simulink model "classic_dtc_final"  (R2026a)
settings: Solver=VariableStepAuto  StopTime=Tsim  MaxStep=1e-6
undefined symbols (not defined in the file): HB_lambda, HB_torque, J, Ki_speed, Kp_speed, lambda_ref, p, Rs, t_load, TL, TL_init, Ts_dtc, Vdc
libraries: nesl_utility x13, fl_lib x10, ee_lib x5, slpidlib x1
settings Model: Creator=kunal  LastModifiedBy=kunal
settings SimscapeCC: SimscapeLogType=none

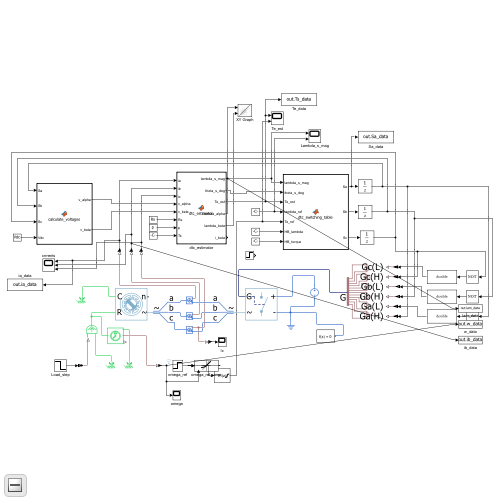
[thumbnail: Simulink's stored preview of the top-level diagram]
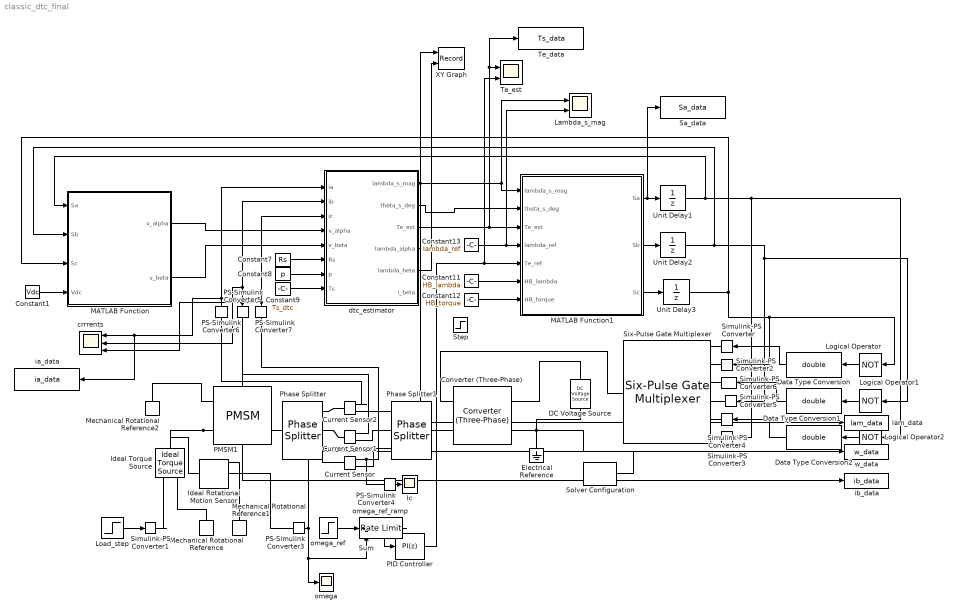
== system classic_dtc_final ==
  Constant1 : Constant  Value=Vdc
  Constant11 : Constant  Value=HB_lambda
  Constant12 : Constant  Value=HB_torque
  Constant13 : Constant  Value=lambda_ref
  Constant7 : Constant  Value=Rs
  Constant8 : Constant  Value=p
  Constant9 : Constant  Value=Ts_dtc
  Converter (Three-Phase) : ee_lib/Semiconductors & Converters/Converters/Converter (Three-Phase)  port_option=ee.enum.threePhasePort.composite  fidelity_option=ee.enum.converters.fidelity.detailed  device_type=ee.enum.converters.switchingdevice.ideal  showThermalPort=false  K=0  Vth=0.5 V  Vgt=1 V  Vgt_off=-1 V  Ih=1 A  Vf=0.8 V  Ron=0.001 Ohm  Rds=0.001 Ohm  Goff=1e-6 1/Ohm  Eon_scalar=22.86e-3 J  Eoff_scalar=17.14e-3 J  Eoff_natural_commutation=10e-3 J  Voff=300 V  Iout_scalar=600 A  onCurrentMeasDelay=0 s  useCurrentFromPreviousCycle=false  useVoltageFromPreviousCycle=false  diode_param=ee.enum.converters.protectiondiode.nodynamics  diode_Vf=0.8 V  diode_Ron=0.001 Ohm  diode_Goff=1e-5 1/Ohm  diode_C=50 nF  diode_iRM=-235 A  diode_iF=300 A  diode_idot=-50 A/us  diode_trr_param=ee.enum.converters.diodetrr.trr_factor  diode_trr_factor=3  diode_trr=15 us  diode_Qrr=1500 s*uA  diode_rec_loss_model=ee.enum.diode.reverseRecoveryModel.fixed  diode_ErecVal=0 J  diode_scaleWithIandV=false  diode_ErecMat=zeros(2, 3) J  diode_TjrecVec=[298.15, 398.15] K  diode_IfrecVec=[.1, 1, 10] A  diode_IrecVal=10 A  diode_VrecVal=10 V  diode_tFilter=1 / 1000 / 100 s  thermal_network_parameterization=ee.enum.thermalNetworkTopology.external  Rth=[.08, .5] K/W  Rth_Cauer=[.08, .1, .5] K/W  Rth_Foster=[.08, .14, .22, .16] K/W  thermal_mass_parameterization=ee.enum.thermalNetwork.timeconstant  thermal_mass=[.01, .5] J/K  thermal_mass_Cauer=[.01, .1, .5] J/K  thermal_mass_Foster=[.001, .005, .05, .5] J/K  thermal_time_constant=[.001, .2] s  thermal_time_constant_Cauer=[.001, .1, .2] s  thermal_time_constant_Foster=[7e-05, .0007, .01, .08] s  thermal_mass_initial_temperatures=[25, 25] degC  thermal_mass_initial_temperatures_Cauer=[25, 25, 25] degC  junction_thermal_mass=0.01 J/K  Tvec_initial_Foster=[25, 25, 25, 25] degC  snubber_type=ee.enum.converters.snubber.exclude  Cs=1e-7 F  Rs=0.1 Ohm  Vce_loss=[0, 150, 300] V
  Current Sensor : fl_lib/Electrical/Electrical Sensors/Current Sensor
  Current Sensor1 : fl_lib/Electrical/Electrical Sensors/Current Sensor
  Current Sensor2 : fl_lib/Electrical/Electrical Sensors/Current Sensor
  DC Voltage Source : fl_lib/Electrical/Electrical Sources/DC Voltage Source  v0=Vdc V
  Data Type Conversion : DataTypeConversion  OutDataTypeStr=double  SaturateOnIntegerOverflow=off  RndMeth=Floor
  Data Type Conversion1 : DataTypeConversion  OutDataTypeStr=double  SaturateOnIntegerOverflow=off  RndMeth=Floor
  Data Type Conversion2 : DataTypeConversion  OutDataTypeStr=double  SaturateOnIntegerOverflow=off  RndMeth=Floor
  Electrical Reference : fl_lib/Electrical/Electrical Elements/Electrical Reference
  Ic : Scope
      settings: ActiveDisplayYMinimum=-1.574268599657235  ActiveDisplayYMaximum=1.0954007787431075  DataLoggingVariableName=ScopeData3
  Ideal Rotational Motion Sensor : fl_lib/Mechanical/Mechanical Sensors/Ideal Rotational Motion Sensor  reference=foundation.enum.MeasurementReference.difference  acceleration_port=false  velocity_port=true  position_port=true  wrap_angle=false  offset=0 rad
  Ideal Torque Source : fl_lib/Mechanical/Mechanical Sources/Ideal Torque Source
  Lambda_s_mag : Scope  NumInputPorts=2
      settings: ActiveDisplayYMinimum=0.17238629365269534  ActiveDisplayYMaximum=0.17761260298821638
  Load_step : Step  Time=t_load  InitialValue=-TL_init  FinalValue=-TL  SampleTime=0
  Logical Operator : Logic  Operator=NOT  AllPortsSameDT=off  OutDataTypeStr=boolean
  Logical Operator1 : Logic  Operator=NOT  AllPortsSameDT=off  OutDataTypeStr=boolean
  Logical Operator2 : Logic  Operator=NOT  AllPortsSameDT=off  OutDataTypeStr=boolean
  MATLAB Function : MATLAB Function  TreatAsAtomicUnit=on  SystemSampleTime=Ts_dtc
  MATLAB Function1 : MATLAB Function  TreatAsAtomicUnit=on  SystemSampleTime=Ts_dtc
  Mechanical Rotational Reference : fl_lib/Mechanical/Rotational Elements/Mechanical Rotational Reference
  Mechanical Rotational Reference1 : fl_lib/Mechanical/Rotational Elements/Mechanical Rotational Reference
  Mechanical Rotational Reference2 : fl_lib/Mechanical/Rotational Elements/Mechanical Rotational Reference
  PID Controller : slpidlib/PID Controller  Controller=PI  Form=Parallel  TimeDomain=Discrete-time  UseExternalTs=off  SampleTime=Ts_dtc  IntegratorMethod=Forward Euler  FilterMethod=Forward Euler  ControllerParametersSource=internal  P=Kp_speed  I=Ki_speed  UseKiTs=off  D=0  UseExternalDerivativeSource=off  N=100  UseFilter=on  TunerSelectOption=Transfer Function Based (PID Tuner App)  InitialConditionSource=internal  InitialConditionForIntegrator=0  InitialConditionForFilter=0  DifferentiatorICPrevScaledInput=0  ExternalReset=none  TrackingMode=off  Kt=1  LimitOutput=on  SatLimitsSource=internal  UpperSaturationLimit=5  LowerSaturationLimit=-5  LinearizeAsGain=on  AntiWindupMode=clamping  Kb=1  LimitIntegrator=off  UpperIntegratorSaturationLimit=inf  LowerIntegratorSaturationLimit=-inf  POutMin=[]  POutMax=[]  IOutMin=[]  IOutMax=[]  DOutMin=[]  DOutMax=[]  NOutMin=[]  NOutMax=[]  SumOutMin=[]  SumOutMax=[]  SaturationOutMin=[]  SaturationOutMax=[]  PParamMin=[]  PParamMax=[]  IParamMin=[]  IParamMax=[]  DParamMin=[]  DParamMax=[]  NParamMin=[]  NParamMax=[]  KbParamMin=[]  KbParamMax=[]  KtParamMin=[]  KtParamMax=[]  KbOutMin=[]  KbOutMax=[]  KtOutMin=[]  KtOutMax=[]  IntegratorOutMin=[]  IntegratorOutMax=[]  FilterOutMin=[]  FilterOutMax=[]  SumI1OutMin=[]  SumI1OutMax=[]  SumI2OutMin=[]  SumI2OutMax=[]  SumI3OutMin=[]  SumI3OutMax=[]  SumI4OutMin=[]  SumI4OutMax=[]  SumDOutMin=[]  SumDOutMax=[]  DifferentiatorOutMin=[]  DifferentiatorOutMax=[]  FilterDiffOutCoefMin=[]  FilterDiffOutCoefMax=[]  ReciprocalOutMin=[]  ReciprocalOutMax=[]  SumDenOutMin=[]  SumDenOutMax=[]  SumNumOutMin=[]  SumNumOutMax=[]  DivideOutMin=[]  DivideOutMax=[]  UdiffTsProdOutMin=[]  UdiffTsProdOutMax=[]  NTsProdOutMin=[]  NTsProdOutMax=[]  UintegralTsProdOutMin=[]  UintegralTsProdOutMax=[]  UngainTsProdOutMin=[]  UngainTsProdOutMax=[]  ClampingZeroOutDataTypeStr=Inherit: Inherit via back propagation  ClampingZeroOutMin=[]  ClampingZeroOutMax=[]  FilterDenConstantOutDataTypeStr=Inherit: Inherit via back propagation  FilterDenConstantOutMin=[]  FilterDenConstantOutMax=[]  PCopyOutDataTypeStr=Inherit: Inherit via back propagation  PCopyOutMin=[]  PCopyOutMax=[]  NCopyOutDataTypeStr=Inherit: Inherit via back propagation  NCopyOutMin=[]  NCopyOutMax=[]  IntegratorContinuousStateAttributes=''  IntegratorStateMustResolveToSignalObject=off  IntegratorRTWStateStorageClass=Auto  FilterContinuousStateAttributes=''  FilterStateMustResolveToSignalObject=off  FilterRTWStateStorageClass=Auto  ParallelPVariant=InternalParameters  IdealPVariant=Disabled  IVariant=InternalParameters  DVariant=Disabled  IntegratorVariant=Discrete  SatVariant=Enabled  AWVariant=DiscClampingParallel  PCopyVariant=Disabled  TRVariant=Disabled  FdbkBlocksVariant=Forward  IdealPFdbkVariant=Disabled  SatFdbkVariant=Disabled  DerivativeFilterVariant=Disabled  NVariant=Disabled  NCopyVariant=Disabled_SignalSpec  FilterICVariant=Disabled  IntegratorICVariant=InternalICs  ExternalResetVariant=Disabled  TRSumVariant=Passthrough  SumFdbkVariant=Disabled  SumVariant=Sum_PI  TsampFilterVariant=InternalTs  TsampNgainVariant=Passthrough  TsampIntegralVariant=Disabled_SignalSpec  ExternalSaturationOutDataTypeStr=Inherit: Same as second input  DerivativeSourceVariant=Disabled  PreIntVariant=InternalPreInt
  PMSM1 : ee_lib/Electromechanical/Permanent Magnet/PMSM  port_option=ee.enum.threePhasePort.composite  winding_type=ee.enum.electromech.statorconfiguration.wye  machine_param=ee.enum.pmsm.parameterization.constant  nPolePairs=p  pmflux_param=ee.enum.pmflux.fluxlinkage  pm_flux_linkage=lambda_f Wb  torque_constant=0.18 N*m/A  back_emf_constant=0.18 V*s/rad  stator_param=ee.enum.statorparam.LdLqL0  Ld=Ld H  Lq=Lq H  idVec=[-200, 0, 200] A  iqVec=[-200, 0, 200] A  LdMatrix=0.0002 * ones(3, 3) H  LqMatrix=0.0002 * ones(3, 3) H  PmMatrix=0.1 * ones(3, 3) Wb  ktMatrix=0.18 * ones(3, 3) N*m/A  keMatrix=0.18 * ones(3, 3) V*s/rad  L0=0.00016 H  Ls=0.0002 H  Lm=-0.00002 H  Ms=0.00002 H  Rs=Rs Ohm  zero_sequence=ee.enum.park.zerosequence.include  axes_param=ee.enum.rotorangle.daxis  loss_param=ee.enum.ironloss.none  losses_oc=[0, 0, 0] W  losses_sc=[0, 0, 0] W  f_losses=60 Hz  Isc_losses=95 A  J=J kg*m^2  lam=B N*m*s/rad  i_d_specify=off  i_d_priority=None  i_d=0 A  i_d_nominal_specify=off  i_d_nominal_value=1  i_d_nominal_unit=A  i_q_specify=off  i_q_priority=None  i_q=0 A  i_q_nominal_specify=off  i_q_nominal_value=1  i_q_nominal_unit=A  torque_specify=off  torque_priority=None  torque=0 N*m  torque_nominal_specify=off  torque_nominal_value=1  torque_nominal_unit=N*m  angular_velocity_specify=off  angular_velocity_priority=High  angular_velocity=0 rpm  angular_velocity_nominal_specify=off  angular_velocity_nominal_value=1  angular_velocity_nominal_unit=rpm  angular_position_specify=off  angular_position_priority=High  angular_position=0 deg  angular_position_nominal_specify=off  angular_position_nominal_value=1  angular_position_nominal_unit=deg  alpha=3.93e-3 1/K  alpha_flux=-0.001 1/K  Tmeas=298.15 K  stator_thermal_mass=100 J/K  rotor_thermal_mass=200 J/K  Rm_percent_rotor=90  Rd_percent_rotor=30  temperatureA_specify=off  temperatureA_priority=High  temperatureA=25 degC  temperatureA_nominal_specify=off  temperatureA_nominal_value=1  temperatureA_nominal_unit=degC  temperatureB_specify=off  temperatureB_priority=High  temperatureB=25 degC  temperatureB_nominal_specify=off  temperatureB_nominal_value=1  temperatureB_nominal_unit=degC  temperatureC_specify=off  temperatureC_priority=High  temperatureC=25 degC  temperatureC_nominal_specify=off  temperatureC_nominal_value=1  temperatureC_nominal_unit=degC  temperatureR_specify=off  temperatureR_priority=High  temperatureR=25 degC  temperatureR_nominal_specify=off  temperatureR_nominal_value=1  temperatureR_nominal_unit=degC
  PS-Simulink Converter{3..7} (5 alike) : nesl_utility/PS-Simulink Converter  PhysicalDomain=network_engine_domain  SubClassName=ps_output  LeftPortType=input  RightPortType=output  PseudoPeriodic=off  Frequencies=[]  VectorFormat=inherit  Unit=inherit  AffineConversion=off
  Phase Splitter : ee_lib/Connectors & References/Phase Splitter
  Phase Splitter1 : ee_lib/Connectors & References/Phase Splitter
  Sa_data : ToWorkspace  VariableName=Sa_data  SaveFormat=Timeseries  SampleTime=-1
  Simulink-PS Converter{,2..6} (6 alike) : nesl_utility/Simulink-PS Converter  PhysicalDomain=network_engine_domain  SubClassName=ps_input  LeftPortType=input  RightPortType=output  PseudoPeriodic=off  Frequencies=[]  NoiseDistribution=none  NoiseParameters=[]  Unit=1  AffineConversion=off  FilteringAndDerivatives=provide  SimscapeFilterOrder=1  InputFilterTimeConstant=0.001  UdotUserProvided=0
  Simulink-PS Converter1 : nesl_utility/Simulink-PS Converter  PhysicalDomain=network_engine_domain  SubClassName=ps_input  LeftPortType=input  RightPortType=output  PseudoPeriodic=off  Frequencies=[]  NoiseDistribution=none  NoiseParameters=[]  Unit=1  AffineConversion=off  FilteringAndDerivatives=filter  SimscapeFilterOrder=1  InputFilterTimeConstant=1e-3  UdotUserProvided=0
  Six-Pulse Gate Multiplexer : ee_lib/Semiconductors & Converters/Converters/Six-Pulse Gate Multiplexer  port_option=ee.enum.controlport.ps
  Solver Configuration : nesl_utility/Solver Configuration  PhysicalDomain=network_engine_domain  SubClassName=solver  LeftPortType=input  RightPortType=generic  Tones=[]  Harmonics=[]  SimulateNoise=off  Profile=off  UseLocalSampling=off  EnableSwitchedLinearOptims=on  FrequencyDomain=off  UseCCode=off  RelTol=0.001  AbsTol=0.001  MinStep=1e-09  ToWorkspace=off  RevertToSquareIcSolve=off  NumHomotopyIterations=100  PhasorMode=off  PhasorModeNumHarmonics=1  ConsistencySolver=NEWTON_XTOL_AFTER_FTOL  CanonicalOrdering=CANONICAL  OptimizeIntermediates=OPTIMIZED  IndexReductionMethod=DerivativeReplacement  DoDC=off  ResidualTolerance=1e-09  ConsistencyTolSource=GLOBAL  ConsistencyAbsTol=0.001  ConsistencyRelTol=0.001  ConsistencyTolFactor=0.001  UseLocalSolver=off  LocalSolverChoice=NE_BACKWARD_EULER_ADVANCER  ResolveIndetEquations=on  FunctionEvalNumThread=1  LocalSolverSampleTime=0.001  DoFixedCost=off  MaxNonlinIter=3  MaxModeIter=2  ComputeImpulses=off  ImpulseIterations=2  LinearAlgebra=auto  LinearAlgebraNumThread=0  EquationFormulation=NE_TIME_EF  DelaysMemoryBudget=1024  AutomaticFiltering=on  FilteringTimeConstant=0.001  PartitionStorageMethod=AS_NEEDED  PartitionMemoryBudget=1024  PartitionMethod=ROBUST  MultibodyUseLocalSolver=off  MultibodyLocalSolverChoice=ODE1  MultibodyLocalSolverSampleTime=0.001
  Step : Step  Time=0.3  FinalValue=0.5  SampleTime=Ts_dtc
  Sum : Sum  Inputs=|+-
  Te_data : ToWorkspace  VariableName=Ts_data  SaveFormat=Timeseries  SampleTime=-1
  Te_est : Scope  NumInputPorts=2
      settings: ActiveDisplayYMinimum=-0.7454839045495818  ActiveDisplayYMaximum=5.7226303419643028
  Unit Delay1 : UnitDelay  SampleTime=Ts_dtc
  Unit Delay2 : UnitDelay  SampleTime=Ts_dtc
  Unit Delay3 : UnitDelay  SampleTime=Ts_dtc
  XY Graph : Record  NumPorts=2.0  FileSettingsInternal="{\"entries\":[{\"content\":{\"excelSettings\":{\"content\":{},\"type\":\"Streamout.ExcelSettings\"},\"parquetSettings\":{\"content\":{},\"type\":\"Streamout.ParquetSettings\"}},\"type\":\"Streamout.FileSettingStorage\",\"uuid\":\"\"}],\"packageUris\":[\"http:\\/\\/schema.mathworks.com\\/mf0\\/streamout_blocks\\/R2020a\"],\"version\":\"1.0\"}"  FrameSettings=[0, 0]  Layout=[1 1]  SignalsInternal="{\"entries\":[{\"content\":{\"signals\":[{\"content\":{\"blockPath\":[],\"dimensions\":[1],\"domain\":\"\",\"lineColor\":\"#edb120\",\"lineWidth\":2,\"port\":1,\"signalID\":1},\"type\":\"RecordBlkView.Signal\",\"uuid\":\"\"},{\"content\":{\"blockPath\":[],\"dimensions\":[1],\"domain\":\"\",\"lineColor\":\"#a2142f\",\"lineWidth\":2,\"plots\":[ 1 ],\"port\":1,\"signalID\":2,\"signalName\":\"dtc_estimator:4\"},\"type\":\"RecordBlkView.Signal\",\"uuid\":\"\"},{\"content\":{\"blockPath\":[],\"dimensions\":[1],\"domain\":\"\",\"lineColor\":\"#4dbeee\",\"lineWidth\":2,\"port\":1,\"signalID\":3,\"signalName\":\"MATLAB Function1:1\"},\"type\":\"RecordBlkView.Signal\",\"uuid\":\"\"},{\"content\":{\"blockPath\":[],\"dimensions\":[1],\"domain\":\"\",\"lineColor\":\"#a2142f\",\"lineWidth\":2,\"port\":1,\"signalID\":4,\"signalName\":\"dtc_estimator:3\"},\"type\":\"RecordBlkView.Signal\",\"uuid\":\"\"},{\"content\":{\"blockPath\":[],\"dimensions\":[1],\"domain\":\"\",\"lineColor\":\"#139fff\",\"lineWidth\":2,\"port\":1,\"signalID\":5,\"signalName\":\"PS-Simulink\\nConverter6\"},\"type\":\"RecordBlkView.Signal\",\"uuid\":\"\"},{\"content\":{\"blockPath\":[],\"dimensions\":[1],\"domain\":\"\",\"lineColor\":\"#139fff\",\"lineWidth\":2,\"plots\":[ 1 ],\"port\":2,\"signalID\":6,\"signalName\":\"dtc_estimator:5\"},\"type\":\"RecordBlkView.Signal\",\"uuid\":\"\"}]},\"type\":\"RecordBlkView.InputSignals\",\"uuid\":\"\"}],\"packageUris\":[\"http:\\/\\/schema.mathworks.com\\/mf0\\/streamout_blocks\\/R2020a\"],\"version\":\"1.0\"}"  VisualizationBindings="{\"xyplotplugin\":{\"info\":[{\"series\":[{\"bindingParametersList\":[{\"parameter\":\"X-Axis\",\"signalID\":6,\"signalName\":\"dtc_estimator:5\"},{\"parameter\":\"Y-Axis\",\"signalID\":2,\"signalName\":\"dtc_estimator:4\"}],\"seriesID\":0}],\"subplotID\":1}]}}"  CompatibilityTag=XY
  crrrents : Scope  NumInputPorts=3
      settings: ActiveDisplayYMinimum=-0.84095457498460979  ActiveDisplayYMaximum=0.85331725762283572  DataLoggingVariableName=ScopeData13
  dtc_estimator : MATLAB Function  TreatAsAtomicUnit=on  SystemSampleTime=Ts_dtc
  ia_data : ToWorkspace  VariableName=ia_data  SaveFormat=Timeseries  SampleTime=-1
  ib_data : ToWorkspace  VariableName=ib_data  SaveFormat=Timeseries  SampleTime=-1
  lam_data : ToWorkspace  VariableName=lam_data  SaveFormat=Timeseries  SampleTime=-1
  omega : Scope
      settings: ActiveDisplayYMinimum=4.4842627024722095  ActiveDisplayYMaximum=29.582290486365775  DataLoggingVariableName=ScopeData2
  omega_ref : Step  Time=0.05  FinalValue=w_ref  SampleTime=Ts_dtc
  omega_ref_ramp : RateLimiter  RisingSlewLimit=700  FallingSlewLimit=-700  SampleTimeMode=inherited
  w_data : ToWorkspace  VariableName=w_data  SaveFormat=Timeseries  SampleTime=-1
  wires:
  Logical Operator2/1 -> Data Type Conversion2/1
  Logical Operator1/1 -> Data Type Conversion1/1
  Constant12/1 -> MATLAB Function1/7(HB_torque)
  Constant7/1 -> dtc_estimator/6(Rs)
  Constant8/1 -> dtc_estimator/7(p)
  MATLAB Function1/3(Sc) -> Unit Delay3/1
  PID Controller/1 -> MATLAB Function1/5(Te_ref), Te_est/2
  Constant11/1 -> MATLAB Function1/6(HB_lambda)
  dtc_estimator/1(lambda_s_mag) -> MATLAB Function1/1(lambda_s_mag), Lambda_s_mag/1, lam_data/1
  MATLAB Function/2(v_beta) -> dtc_estimator/5(v_beta)
  MATLAB Function1/2(Sb) -> Unit Delay2/1
  dtc_estimator/2(theta_s_deg) -> MATLAB Function1/2(theta_s_deg)
  MATLAB Function/1(v_alpha) -> dtc_estimator/4(v_alpha)
  Logical Operator/1 -> Data Type Conversion/1
  dtc_estimator/3(Te_est) -> Te_data/1, Te_est/1, MATLAB Function1/3(Te_est)
  Constant9/1 -> dtc_estimator/8(Ts)
  Constant13/1 -> Lambda_s_mag/2, MATLAB Function1/4(lambda_ref)
  Data Type Conversion/1 -> Simulink-PS Converter/1
  Unit Delay1/1 -> Logical Operator2/1, Simulink-PS Converter3/1, MATLAB Function/1(Sa)
  Unit Delay3/1 -> Logical Operator/1, Simulink-PS Converter2/1, MATLAB Function/3(Sc)
  PS-Simulink Converter3/1 -> Sum/2, omega/1, w_data/1
  PS-Simulink Converter4/1 -> Ic/1
  Unit Delay2/1 -> MATLAB Function/2(Sb), Simulink-PS Converter5/1, Logical Operator1/1
  Constant1/1 -> MATLAB Function/4(Vdc)
  PS-Simulink Converter5/1 -> crrrents/2, dtc_estimator/2(ib), ib_data/1
  PS-Simulink Converter7/1 -> dtc_estimator/3(ic), crrrents/3
  Data Type Conversion2/1 -> Simulink-PS Converter4/1
  Data Type Conversion1/1 -> Simulink-PS Converter6/1
  PS-Simulink Converter6/1 -> ia_data/1, crrrents/1, dtc_estimator/1(ia)
  dtc_estimator/4(lambda_alpha) -> XY Graph/1
  dtc_estimator/5(lambda_beta) -> XY Graph/2
  MATLAB Function1/1(Sa) -> Sa_data/1, Unit Delay1/1
  Sum/1 -> PID Controller/1
  omega_ref/1 -> omega_ref_ramp/1
  omega_ref_ramp/1 -> Sum/1
  Load_step/1 -> Simulink-PS Converter1/1
  connections:
  Electrical Reference/LConn1 -- Solver Configuration/RConn1 -- Converter (Three-Phase)/RConn2 -- DC Voltage Source/RConn1
  PMSM1/RConn1 -- Ideal Rotational Motion Sensor/LConn1 -- Ideal Torque Source/LConn1
  Phase Splitter/RConn2 -- Current Sensor1/LConn1
  Phase Splitter1/RConn2 -- Current Sensor1/RConn2
  Current Sensor/RConn1 -- PS-Simulink Converter7/LConn1 -- PS-Simulink Converter4/LConn1
  Current Sensor2/RConn2 -- Phase Splitter1/RConn1
  Simulink-PS Converter4/RConn1 -- Six-Pulse Gate Multiplexer/LConn2
  Simulink-PS Converter6/RConn1 -- Six-Pulse Gate Multiplexer/LConn4
  Phase Splitter1/RConn3 -- Current Sensor/RConn2
  Simulink-PS Converter5/RConn1 -- Six-Pulse Gate Multiplexer/LConn3
  Simulink-PS Converter/RConn1 -- Six-Pulse Gate Multiplexer/LConn6
  Phase Splitter/RConn3 -- Current Sensor/LConn1
  Converter (Three-Phase)/LConn2 -- Phase Splitter1/LConn1
  Simulink-PS Converter3/RConn1 -- Six-Pulse Gate Multiplexer/LConn1
  Simulink-PS Converter1/RConn1 -- Ideal Torque Source/RConn1
  Simulink-PS Converter2/RConn1 -- Six-Pulse Gate Multiplexer/LConn5
  Current Sensor2/LConn1 -- Phase Splitter/RConn1
  Six-Pulse Gate Multiplexer/RConn1 -- Converter (Three-Phase)/LConn1
  PMSM1/LConn1 -- Phase Splitter/LConn1
  Mechanical Rotational Reference/LConn1 -- Ideal Torque Source/RConn2
  Converter (Three-Phase)/RConn1 -- DC Voltage Source/LConn1
  Mechanical Rotational Reference2/LConn1 -- PMSM1/RConn2
  Ideal Rotational Motion Sensor/RConn2 -- PS-Simulink Converter3/LConn1
  Current Sensor2/RConn1 -- PS-Simulink Converter6/LConn1
  Current Sensor1/RConn1 -- PS-Simulink Converter5/LConn1
  Ideal Rotational Motion Sensor/RConn1 -- Mechanical Rotational Reference1/LConn1

== matlab function classic_dtc_final/MATLAB Function1 ==
  data: lambda_s_mag input; Sa output; theta_s_deg input; Te_est input; lambda_ref input; Te_ref input; HB_lambda input; HB_torque input; Sb output; Sc output
function [Sa, Sb, Sc] = dtc_switching_table(lambda_s_mag, theta_s_deg, Te_est, ...
    lambda_ref, Te_ref, HB_lambda, HB_torque)
%#codegen
% DTC hysteresis comparators + switching table (Parts 4.4-4.6)
% Outputs the 3-phase switching state (Sa,Sb,Sc) each in {0,1}
% Feed this into a Simulink "Controlled Voltage Source" / averaged VSI
% block, or directly into a full switched IGBT bridge if you're doing
% detailed power-electronics simulation.

persistent d_lambda d_torque
if isempty(d_lambda)
    d_lambda = 1;   % start assuming flux needs to rise
    d_torque = 0;
end

%% --- Flux hysteresis comparator (2-level, Part 4.4) ---
flux_err = lambda_ref - lambda_s_mag;
if flux_err > HB_lambda
    d_lambda = 1;
elseif flux_err < -HB_lambda
    d_lambda = 0;
end
% else: hold previous value (hysteresis behavior)

%% --- Torque hysteresis comparator (3-level, Part 4.4) ---
torque_err = Te_ref - Te_est;
if torque_err > HB_torque
    d_torque = 1;
elseif torque_err < -HB_torque
    d_torque = -1;
else
    d_torque = 0;
end

%% --- Sector identification (Step 1 from the sector clarification) ---
theta = mod(theta_s_deg, 360);
if theta >= 330 || theta < 30
    n = 1;
elseif theta < 90
    n = 2;
elseif theta < 150
    n = 3;
elseif theta < 210
    n = 4;
elseif theta < 270
    n = 5;
else
    n = 6;
end

%% --- Vector selection rule (Step 2 from the sector clarification) ---
% Vector index wraps mod 6, mapped to 1-6 (no zero index)
wrap6 = @(k) mod(k-1,6) + 1;

if d_torque == 0
    vec_idx = 0;   % zero vector (alternate V0/V7 for switching loss balance)
elseif d_lambda == 1 && d_torque == 1
    vec_idx = wrap6(n+1);
elseif d_lambda == 1 && d_torque == -1
    vec_idx = wrap6(n-1);
elseif d_lambda == 0 && d_torque == 1
    vec_idx = wrap6(n+2);
else % d_lambda == 0 && d_torque == -1
    vec_idx = wrap6(n-2);
end

%% --- Map vector index to switching state (Part 3.2 table) ---
switch vec_idx
    case 0
        Sa = 0; Sb = 0; Sc = 0;     % V0 (use V7=[1 1 1] on alternating cycles)
    case 1
        Sa = 1; Sb = 0; Sc = 0;     % V1
    case 2
        Sa = 1; Sb = 1; Sc = 0;     % V2
    case 3
        Sa = 0; Sb = 1; Sc = 0;     % V3
    case 4
        Sa = 0; Sb = 1; Sc = 1;     % V4
    case 5
        Sa = 0; Sb = 0; Sc = 1;     % V5
    case 6
        Sa = 1; Sb = 0; Sc = 1;     % V6
    otherwise
        % Should be unreachable given vec_idx is always 0-6, but
        % MATLAB Coder requires every output defined on every path.
        Sa = 0; Sb = 0; Sc = 0;
end

end

== matlab function classic_dtc_final/dtc_estimator ==
  settings: updateMethod=DISCRETE
  data: ia input; lambda_s_mag output; ib input; ic input; v_alpha input; v_beta input; Rs input; p input; Ts input; theta_s_deg output; Te_est output; lambda_alpha output; lambda_beta output; i_beta output
function [lambda_s_mag, theta_s_deg, Te_est, lambda_alpha, lambda_beta, i_beta] = dtc_estimator(ia, ib, ic, v_alpha, v_beta, Rs, p, Ts)
%#codegen
% DTC flux and torque estimator (voltage model, Part 4.3)
% Implements this as a MATLAB Function block with two persistent
% integrator states (lambda_alpha, lambda_beta).
%
% Inputs:
%   ia, ib, ic      - measured phase currents [A]
%   v_alpha, v_beta - inverter output voltage in alpha-beta frame [V]
%                     (computed upstream from the switching state, Part 3.2)
%   Rs              - stator resistance [ohm]
%   p               - pole pairs
%   Ts              - sample time [s]
%
% Outputs:
%   lambda_s_mag - stator flux magnitude [Wb]
%   theta_s_deg  - stator flux angle [deg], wrapped to [0,360)
%   Te_est       - estimated electromagnetic torque [N*m]
%   lambda_alpha, lambda_beta - flux components, useful for scope/debug

%{
This is the block that answers the two questions torque control actually depends on: how big is my stator flux, and what angle is it 
at relative to where it started — recall from Part 4.2, torque depends on the angle between stator flux and rotor flux, 
and this angle is embedded in how theta_s_deg evolves over time.
%}


persistent lam_a lam_b
if isempty(lam_a)
    lam_a = 0.175;
    lam_b = 0;
end
%% Correct physical current inversion from the sensors
ia_true = -ia;
ib_true = -ib;

%% Clarke transform of true currents
i_alpha = ia_true;
i_beta  = (1/sqrt(3))*ia_true + (2/sqrt(3))*ib_true;

%% Flux integration (Part 4.3) — forward Euler, simplest form
% NOTE: pure integration drifts at low speed (Problem 3, Part 5.1).
% Once this base version works, replace with a low-pass-filter-based
% or closed-loop observer estimator and compare.
lam_a = lam_a + Ts * (v_alpha - Rs*i_alpha);
lam_b = lam_b + Ts * (v_beta  - Rs*i_beta);


lambda_alpha = lam_a;
lambda_beta  = lam_b;

%% Magnitude and angle
lambda_s_mag = sqrt(lam_a^2 + lam_b^2);
theta_s_rad  = atan2(lam_b, lam_a);
theta_s_deg  = mod(theta_s_rad * 180/pi, 360);

%% Torque estimate (Part 4.3)
Te_est = 1.5 * p * (lam_a*i_beta - lam_b*i_alpha);

end

== matlab function classic_dtc_final/MATLAB Function ==
  data: Sa input; v_alpha output; Sb input; Sc input; Vdc input; v_beta output
function [v_alpha, v_beta] = calculate_voltages(Sa, Sb, Sc, Vdc)
% Calculate alpha-beta voltages based on switching states and DC link
v_alpha = (2/3) * Vdc * (Sa - 0.5 * (Sb + Sc));
v_beta  = (2/3) * Vdc * (sqrt(3)/2) * (Sb - Sc);
end

%{
Inputs: Sa, Sb, Sc (the switching state chosen last cycle), Vdc
Outputs: v_alpha, v_beta

This answers: given the switch positions I already commanded, what voltage is actually sitting on the motor terminals right now? 
It doesn't measure anything — it's a pure calculation from Part 3.2's formula, because a 2-level inverter's output voltage is fully determined by which switches are on. 
This is one of the things that makes DTC elegant: you never need a voltage sensor, just knowledge of your own last command plus Vdc.

This feeds straight into the estimator, because the estimator needs to know "how much voltage pushed the flux where it is now."
%}
